simulink library "aeroelasticity_lib"  (R2018b)
settings: Solver=VariableStepAuto  StartTime=0.0  StopTime=10.0  RelTol=1e-3
undefined symbols (not defined in the file or in its folder): structure, structure_red, structureGetBendingMomentTrafoAt, structureGetCutLoadTrafoAt, wing_main, wingAeroelasticityGetGravityLoading, wingGetBendingMoment
settings Model: Creator=Ybeyer  LastModifiedBy=yannic
settings SFSimCC: SimUseLocalCustomCode=off
settings RTWCC: RTWUseLocalCustomCode=off
settings CodeAppCC: StateflowObjectComments=on

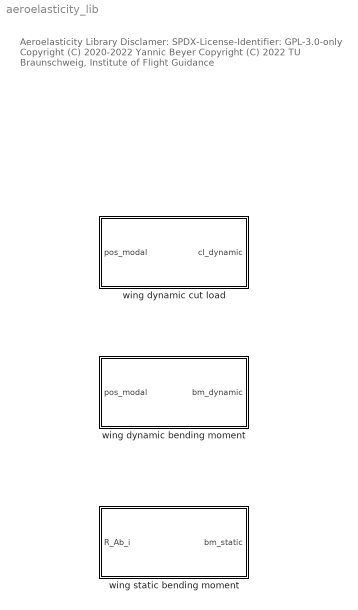
== system aeroelasticity_lib ==
  note: Aeroelasticity Library
      |
      | Disclamer:
      | SPDX-License-Identifier: GPL-3.0-only
      |
      | Copyright (C) 2020-2022 Yannic Beyer
      | Copyright (C) 2022 TU Braunschweig, Institute of Flight Guidance
  wing dynamic bending moment : Subsystem  mask{structure=structure, structure_red=structure_red, eta=[-0.9:0.2:0.9]}
      mask prompts: structure "structure struct"; structure_red "reduced order structure struct"; eta "dimensionless spanwise positions"
      mask DialogControl DescGroupVar Prompt: Wing dynamic bending moment
      mask DialogControl DescTextVar Prompt: Compute dynamic bending moment at specified dimensionless spanwise positions.
      mask DialogControl Control3 Prompt: The dynamic loading considers the internal forces of the reduced order structure due to the displacements.
      mask DialogControl Control2 Prompt: Note that the order of the reduced order structural model must be sufficiently high in order to get accurate absolute values.
  wing dynamic cut load : Subsystem  mask{structure=structure, structure_red=structure_red, eta=[-0.9:0.2:0.9], popup_index_1=Mx, popup_index_2=reverse_none}
      mask prompts: structure "structure struct"; structure_red "reduced order structure struct"; eta "dimensionless spanwise positions"; popup_index_1 "load type"; popup_index_2 "reverse sign for wing side"
      mask init:
      | switch popup_index_1
      |     case 1
      |         load_type = 'Mx';
      |     case 2
      |         load_type = 'My';
      |     case 3
      |         load_type = 'Mz';
      |     case 4
      |         load_type = 'Fx';
      |     case 5
      |         load_type = 'Fy';
      |     case 6
      |         load_type = 'Fz';
      |     case 7
      |         load_type = 'all';
      | end
      | 
      | switch popup_index_2
      |     case 1
      |         reverse_side = 'reverse_none';
      |     case 2
      |         reverse_side = 'reverse_left';
      |     case 3
      |         reverse_side = 'reverse_right';
      | end
      mask TypeOptions popup_index_1: Mx | My | Mz | Fx | Fy | Fz | all
      mask TypeOptions popup_index_2: reverse_none | reverse_left | reverse_right
      mask DialogControl DescGroupVar Prompt: Wing dynamic cut load
      mask DialogControl DescTextVar Prompt: Compute transformation matrix from generalized structure positions to dynamic cut load at specified dimensionless spanwise positions.
      mask DialogControl Control3 Prompt: The dynamic loading considers the internal forces and moments of the reduced order structure due to the displacements.
      mask DialogControl Control2 Prompt: Note that the order of the reduced order structural model must be sufficiently high in order to get accurate absolute values.
  wing static bending moment : Subsystem  mask{wing_main=wing_main, structure=structure, eta=[-0.9:0.2:0.9]}
      mask prompts: wing_main "wing struct"; structure "structure struct"; eta "dimensionless spanwise positions"
      mask DialogControl DescGroupVar Prompt: Wing static bending moment
      mask DialogControl DescTextVar Prompt: Compute static bending moment at specified dimensionless spanwise positions.
      mask DialogControl Control2 Prompt: The static loading considers both the aerodynamic forces and the static gravitational forces.

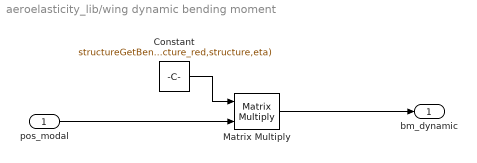
== system aeroelasticity_lib/wing dynamic bending moment ==
  pos_modal : Inport
  Constant : Constant  Value=structureGetBendingMomentTrafoAt(structure_red,structure,eta)
  Matrix Multiply : Product  Multiplication=Matrix(*)
  bm_dynamic : Outport
  wires:
  Constant/1 -> Matrix Multiply/1
  pos_modal/1 -> Matrix Multiply/2
  Matrix Multiply/1 -> bm_dynamic/1

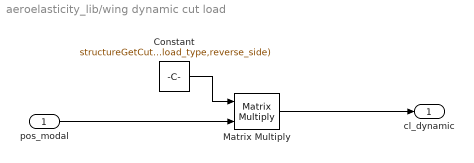
== system aeroelasticity_lib/wing dynamic cut load ==
  pos_modal : Inport
  Constant : Constant  Value=structureGetCutLoadTrafoAt(structure_red,structure,eta,load_type,reverse_side)
  Matrix Multiply : Product  Multiplication=Matrix(*)
  cl_dynamic : Outport
  wires:
  Matrix Multiply/1 -> cl_dynamic/1
  pos_modal/1 -> Matrix Multiply/2
  Constant/1 -> Matrix Multiply/1

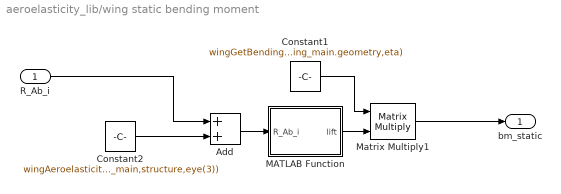
== system aeroelasticity_lib/wing static bending moment ==
  R_Ab_i : Inport
  Add : Sum
  Constant1 : Constant  Value=wingGetBendingMoment(wing_main.geometry,eta)
  Constant2 : Constant  Value=wingAeroelasticityGetGravityLoading(wing_main,structure,eye(3))
  MATLAB Function : MATLAB Function  TreatAsAtomicUnit=on
  Matrix Multiply1 : Product  Multiplication=Matrix(*)
  bm_static : Outport
  wires:
  Constant2/1 -> Add/2
  MATLAB Function/1(lift) -> Matrix Multiply1/2
  Constant1/1 -> Matrix Multiply1/1
  Add/1 -> MATLAB Function/1(R_Ab_i)
  Matrix Multiply1/1 -> bm_static/1
  R_Ab_i/1 -> Add/1

== matlab function aeroelasticity_lib/wing static bending moment/MATLAB Function ==
  data: R_Ab_i input; lift output
function lift = fcn(R_Ab_i)

lift = vecnorm( R_Ab_i(3,:), 2, 1 )';

end
